simulink model "Bossi_Emanuele_EE460S3D_R99"  (R2025a)
settings: Solver=FixedStepDiscrete  StartTime=0.0  StopTime=120  FixedStep=dt0  RelTol=1e-3  EnableMultiTasking=on
PostLoadFcn:
  | %Set the size for the model
  | set_param(gcs,'Location',[10 10 1270 970])
  | %Set the zoom factor for the model
  | set_param(gcs,'ZoomFactor','100')
InitFcn:
  | tic
  | Bossi_Emanuele_EE460_Final
  | INIT_S3D_01
StartFcn:
  | tend0=toc;
  | tic;
StopFcn:
  | tend=toc;
  | disp(['Simulation time = ' num2str(tout(end)) ' sec'])
  | disp(['Real time = ' num2str(tend) ' sec'])
  | title('DONE')
  | SCORE=round((max(0,120-tout(end)-tend0))*4+10*(40-FuelBurned)+sum(100*double(PDONE)-100*double(PDONE<.5)));
  | PlotS3D(PlotInput);
  | text(15,22,['S: ' num2str(SCORE)]);
  | % Reset color scheme back to normal defaults
  | figure()
  | blkwhitebg('w');
  | close
values from neighbouring files (symbols this model uses):
  A_obs = [ 0  1  0  0  0  0 ... (first row only)    [Bossi_Emanuele_EE460_Final.m]
  B_obs = [ 0     0     0 ... (first row only)    [Bossi_Emanuele_EE460_Final.m]
  C_obs = [ 1 0 0 0 0 0 ... (first row only)    [Bossi_Emanuele_EE460_Final.m]
  d2r = pi/180    (= 0.0174532925199)    [INIT_S3D_01.m]
  D_obs = [ 0     0     0 ... (first row only)    [Bossi_Emanuele_EE460_Final.m]
  dt = 0.01    [INIT_S3D_01.m]
  dt0 = 0.001    [INIT_S3D_01.m]
  fr = 100    [INIT_S3D_01.m]
  G = [1,  1, -1, -1,  0,  0,  0,  0 ... (first row only)    [Bossi_Emanuele_EE460_Final.m]
  G_obs = eye(6)    [Bossi_Emanuele_EE460_Final.m]
  HM_S = 250    [INIT_S3D_01.m]
  HM_U = 500    [INIT_S3D_01.m]
  J = Jbase+JC0+JF+M*(Xcg^2+Ycg^2)    [INIT_S3D_01.m]
  Jbase = JC1+4*Ja+2*Ma*da^2+2*Ma*db^2    [INIT_S3D_01.m]
  JC0 = MC0/2    (= 10.2101761242)    [INIT_S3D_01.m]
  Kdtheta = 2 * zeta_th * wn_th * J_eff    [Bossi_Emanuele_EE460_Final.m]
  Kdtheta_fail = 2 * zeta_th_fail * wn_th_fail * J_eff    [Bossi_Emanuele_EE460_Final.m]
  Kdx = 2 * zeta_xy * wn_xy * M_eff    [Bossi_Emanuele_EE460_Final.m]
  Kdx_fail = 2 * zeta_xy_fail * wn_xy_fail * M_eff    [Bossi_Emanuele_EE460_Final.m]
  Kdy = 2 * zeta_xy * wn_xy * M_eff    [Bossi_Emanuele_EE460_Final.m]
  Kdy_fail = 2 * zeta_xy_fail * wn_xy_fail * M_eff    [Bossi_Emanuele_EE460_Final.m]
  Kptheta = J_eff * wn_th^2    [Bossi_Emanuele_EE460_Final.m]
  Kptheta_fail = J_eff * wn_th_fail^2    [Bossi_Emanuele_EE460_Final.m]
  Kpx = M_eff * wn_xy^2    [Bossi_Emanuele_EE460_Final.m]
  Kpx_fail = M_eff * wn_xy_fail^2    [Bossi_Emanuele_EE460_Final.m]
  Kpy = M_eff * wn_xy^2    [Bossi_Emanuele_EE460_Final.m]
  Kpy_fail = M_eff * wn_xy_fail^2    [Bossi_Emanuele_EE460_Final.m]
  L13 = sqrt(10)    [INIT_S3D_01.m]
  L24 = sqrt(6.25)    [INIT_S3D_01.m]
  LVL = LVL12    [INIT_S3D_01.m]
  M = MC+M1+M2+M3+M4+4*Ma    [INIT_S3D_01.m]
  M1 = LVL.M1    [INIT_S3D_01.m]
  M2 = LVL.M2    [INIT_S3D_01.m]
  M3 = LVL.M3    [INIT_S3D_01.m]
  M4 = LVL.M4    [INIT_S3D_01.m]
  max_qddot = [max_qddot_x; max_qddot_y; max_qddot_theta]    [Bossi_Emanuele_EE460_Final.m]
  mdti = (1/300)    (= 0.00333333333333)    [INIT_S3D_01.m]
  P = [1  1 -1 -1  0  0  0  0 ... (first row only)    [Bossi_Emanuele_EE460_Final.m]
  Pdata = [LVL.P1 LVL.P2 LVL.P3 LVL.P4]    [INIT_S3D_01.m]    (also in PlotS3D.m = R*[xt1;yt1+[0 3*tt*TV(idx-13)*TSIG(idx-13) 0]])
  PTvec = [Pdata(:,1);Pdata(:,2);Pdata(:,3);Pdata(:,4) ... (first row only)    [INIT_S3D_01.m]
  Q_obs = eye(6)    [Bossi_Emanuele_EE460_Final.m]
  r2d = 180/pi    (= 57.2957795131)    [INIT_S3D_01.m]
  r_bang = 0.5    [Bossi_Emanuele_EE460_Final.m]
  Sconfig = 1    [Bossi_Emanuele_EE460_Final.m]
  SLIM = [-100 100 ... (first row only)    [INIT_S3D_01.m]
  SQ = [.005 .01 .004 .005 .01 .004 .02 .01 .4]'    [INIT_S3D_01.m]
  SSF = 1./SQ    [INIT_S3D_01.m]
  tau = 0.5    [Bossi_Emanuele_EE460_Final.m]
  TOLdata = [LVL.P1tol LVL.P2tol LVL.P3tol LVL.P4tol]    [INIT_S3D_01.m]
  ULIM = [[Umin Umax];0 0;0 0]    [INIT_S3D_01.m]
undefined symbols (not defined in the file or in its folder): den_lp, den_lp2, DiscIntNeverNeededParam, dt1_bang_3, dt2_bang_3, dtc_bang_3, num_lp, num_lp2, q0_1
libraries: simulink x87, matrix_library x4, sl3dlib x1, aerolibutil x1, aerolibanimutils x1
(part 1 of 8)
settings Model: Creator=bordignk  LastModifiedBy=emab0
settings SolverCC: AlgebraicLoopSolver=TrustRegion
settings DataIOCC: LimitDataPoints=on  SaveFormat=Array  ReturnWorkspaceOutputs=off
settings OptimizationCC: LifeSpan=inf
settings DebuggingCC: CheckSSInitialOutputMsg=off  UnderspecifiedInitializationDetection=Classic  MergeDetectMultiDrivingBlocksExec=none  InheritedTsInSrcMsg=none  ParameterPrecisionLossMsg=none  AllowSymbolicDim=off  StateNameClashWarn=warning  SFUnexpectedBacktrackingDiag=warning  SFNoUnconditionalDefaultTransitionDiag=warning  SFExecutionAtInitializationDiag=none  ArithmeticOperatorsInVariantConditions=warning
settings HardwareCC: ProdBitPerPointer=32.0  ProdBitPerSizeT=32.0  ProdBitPerPtrDiffT=32.0  ProdLargestAtomicFloat=None  ProdIntDivRoundTo=Undefined  ProdEndianess=Unspecified  ProdWordSize=32.0  ProdHWDeviceType=32-bit Generic
settings ModelReferenceCC: EnableRefExpFcnMdlSchedulingChecks=on  PropagateSignalLabelsOutOfModel=off
settings SFSimCC: SimUseLocalCustomCode=off  CustomCodeUndefinedFunction=UseInterfaceOnly
settings RTWCC: RTWUseLocalCustomCode=off  GPUComputeCapability=3.5  DLArmComputeVersion=19.05
settings CodeAppCC: StateflowObjectComments=on
settings GRTTargetCC: TargetLangStandard=C89/C90 (ANSI)
settings ConfigComp: CovMetricSettings=dw  CovSaveCumulativeToWorkspaceVar=on  CovSaveSingleToWorkspaceVar=on  CovExternalEMLEnable=off

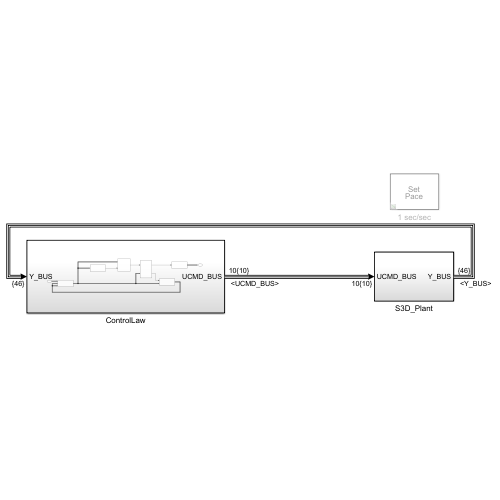
[thumbnail: Simulink's stored preview of the top-level diagram]
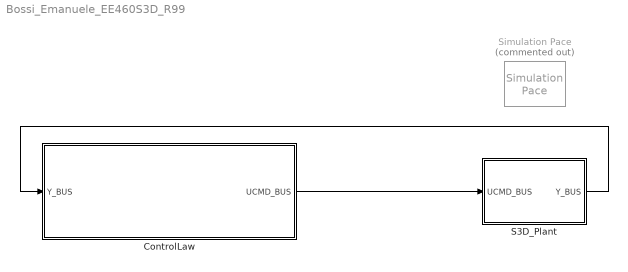
== system Bossi_Emanuele_EE460S3D_R99 ==
  ControlLaw : Subsystem
  S3D_Plant : Subsystem
  Simulation Pace : aerolibanimutils/Simulation Pace  Commented=on  SimulationPace=1  SleepMode=MATLAB Thread  OutputPaceError=off  SampleTime=-1
      settings: AttributesFormatString=%<SimulationPace> sec/sec
  wires:
  S3D_Plant/1(Y_BUS) -> ControlLaw/1(Y_BUS)
  ControlLaw/1(UCMD_BUS) -> S3D_Plant/1(UCMD_BUS)

== system Bossi_Emanuele_EE460S3D_R99/ControlLaw ==
  Y_BUS : Inport
  Command : Subsystem
  ControlAllocation : Subsystem
  InputDataConditioning : Subsystem
  Observer : Subsystem
  OutputDataConditioning : Subsystem
  Regulator : Subsystem
  UCMD_BUS : Outport
  wires:
  OutputDataConditioning/1(UCMD_BUS) -> UCMD_BUS/1
  Y_BUS/1 -> InputDataConditioning/1(Y_BUS)
  ControlAllocation/1(U_lim) -> OutputDataConditioning/1(U_lim)
  Regulator/1(uP_cmd) -> ControlAllocation/1(uP_cmd)
  InputDataConditioning/1(Y_IN) -> Observer/2(Y_IN), ControlAllocation/2(Y_IN), Regulator/1(Y_IN), Command/1(Y_IN)
  ControlAllocation/2(CAout) -> Observer/1(CAout)  "CAout"
  Observer/1(xhat) -> InputDataConditioning/3(xhat_2), InputDataConditioning/2(xhat)  "xhat"
  Command/1(CMD) -> Regulator/2(CMD)  "CMD"

== system Bossi_Emanuele_EE460S3D_R99/S3D_Plant ==
  UCMD_BUS : Inport
  Comm : Subsystem
  GetAccel : Subsystem
  Integrate : Subsystem
  MassProperties : Subsystem
  OutputDataProcessing : Subsystem
  Sensors : Subsystem
  ThrusterValues : Subsystem
  Y_BUS : Outport
  wires:
  Integrate/1(XCentroid) -> OutputDataProcessing/4(x), Comm/1(X), Sensors/1(X), GetAccel/3(X)
  MassProperties/1(MP) -> OutputDataProcessing/1(MP), Integrate/1(MP), GetAccel/1(MP), ThrusterValues/1(MP)
  OutputDataProcessing/1(Y_BUS) -> Y_BUS/1
  Comm/1(COMM) -> OutputDataProcessing/3(COMM)
  Sensors/1(Sensors) -> OutputDataProcessing/2(Sensors)
  ThrusterValues/1(U) -> MassProperties/1(U), OutputDataProcessing/5(U), GetAccel/2(U)
  GetAccel/1(ACCEL) -> Integrate/2(ACCEL)
  UCMD_BUS/1 -> ThrusterValues/2(UCMD_BUS)

== system Bossi_Emanuele_EE460S3D_R99/ControlLaw/Command ==
  Y_IN : Inport
  AutoMode : Subsystem  TreatAsAtomicUnit=on
  Bus Creator : BusCreator  Inputs=6
  Bus Selector : BusSelector  OutputSignals=ManualMode,AutoON,ManualON
  Bus Selector1 : BusSelector  OutputSignals=PointToGo
  Bus Selector2 : BusSelector  OutputSignals=ManualInput
  Bus Selector3 : BusSelector  OutputSignals=Y_IN
  Bus Selector4 : BusSelector  OutputSignals=AutoON,Y_IN
  Bus Selector5 : BusSelector  OutputSignals=ManualMode,Y_IN
  If1 : If  NumInputs=3  IfExpression=u1 == 0 & u2 == 0 & u3 == 0  ElseIfExpressions="(u2  ~= 0 | u3  ~= 0) & u1 == 0"
  InitialPoint : Subsystem  TreatAsAtomicUnit=on
  Joystick : Subsystem
  ManualMode : Subsystem  TreatAsAtomicUnit=on
  Merge : Merge  Inputs=3
  Trigger1 : Subsystem
  Trigger2 : Subsystem
  CMD : Outport
  wires:
  Joystick/1(Out2) -> Bus Creator/1
  Joystick/3(Out4) -> Bus Creator/3  "ManualInput"
  Y_IN/1 -> Bus Creator/6, Joystick/1(Y_IN)
  Joystick/2(Out3) -> Bus Creator/2
  Bus Creator/1 -> Bus Selector2/1, Bus Selector5/1, Bus Selector3/1, Bus Selector1/1, Bus Selector/1, Bus Selector4/1
  Bus Selector1/1 -> AutoMode/1(In2)  "<PointToGo>"
  Merge/1 -> CMD/1  "CMD"
  Bus Selector2/1 -> ManualMode/1(ManualInput)  "<ManualInput>"
  Joystick/4(Out1) -> Bus Creator/4
  ManualMode/1(Out1) -> Merge/3
  AutoMode/1(Out1) -> Merge/2  "CMD"
  InitialPoint/1(Out2) -> Merge/1  "CMD"
  If1/1 -> InitialPoint/Action
  If1/2 -> AutoMode/Action
  If1/3 -> ManualMode/Action
  Bus Selector3/1 -> AutoMode/2(In1)  "<Y_IN>"
  Joystick/5(Out5) -> Bus Creator/5
  Bus Selector/1 -> If1/1  "<ManualMode>"
  Bus Selector/2 -> If1/2  "<AutoON>"
  Bus Selector/3 -> If1/3  "<ManualON>"
  Trigger1/2(Out1) -> InitialPoint/2(In2)
  Bus Selector4/2 -> Trigger1/2(In1)  "<Y_IN>"
  Trigger1/1(Trigger) -> InitialPoint/1(Trigger)
  Bus Selector4/1 -> Trigger1/1(In2)  "<AutoON>"
  Bus Selector5/1 -> Trigger2/1(In2)  "<ManualMode>"
  Bus Selector5/2 -> Trigger2/2(In1)  "<Y_IN>"
  Trigger2/1(Trigger) -> ManualMode/2(Trigger)
  Trigger2/2(TriggeredPosition) -> ManualMode/3(CurrentPosition)
  Trigger2/3(TriggeredVelocity) -> ManualMode/4(CurrentVelocity)

== system Bossi_Emanuele_EE460S3D_R99/ControlLaw/ControlAllocation ==
  uP_cmd : Inport
  Y_IN : Inport  Port=2
  A : Subsystem
  BodyAxisModeling : Subsystem
  Bus Creator : BusCreator  Inputs=2
  Bus Creator1 : BusCreator  Inputs=3
  Bus Selector : BusSelector  OutputSignals=theta_pos_deg
  Bus Selector1 : BusSelector  OutputSignals=R,u_body
  Bus Selector2 : BusSelector  OutputSignals=Failures
  Bus Selector3 : BusSelector  OutputSignals=2A
  Bus Selector4 : BusSelector  OutputSignals=Ufail_mod
  Gain : Gain  Gain=G  Multiplication=Matrix(K*u)
  MatrixMultiply : Product  Multiplication=Matrix(*)
  MatrixMultiply2 : Product  Multiplication=Matrix(*)
  R_theta : Subsystem
  Saturation : Saturate  UpperLimit=100  LowerLimit=0
  Sum : Sum  Inputs=-+|
  Sum1 : Sum  Inputs=++|
  ThrusterFailure : Subsystem
  deg2rad_gain : Gain  Gain=pi/180
  U_lim : Outport  PortDimensions=8
  CAout : Outport  Port=2
  wires:
  MatrixMultiply2/1 -> Sum1/2  "U_mat"
  Saturation/1 -> Gain/1, U_lim/1  "U_lim"
  uP_cmd/1 -> BodyAxisModeling/1(uP_cmd)
  Bus Selector/1 -> deg2rad_gain/1  "<theta_pos_deg>"
  deg2rad_gain/1 -> R_theta/1(In2), BodyAxisModeling/2(theta_rad)  "theta_pos_rad"
  BodyAxisModeling/1(Out1) -> Sum/2  "uP_body"
  MatrixMultiply/1 -> CAout/1  "CAOut"
  R_theta/1(Out1) -> Bus Creator/2  "R"
  Gain/1 -> Bus Creator/1  "u_body"
  Bus Creator/1 -> Bus Selector1/1
  Bus Selector1/1 -> MatrixMultiply/1  "<R>"
  Bus Selector1/2 -> MatrixMultiply/2  "<u_body>"
  Y_IN/1 -> Bus Selector/1, A/1(Y_IN), ThrusterFailure/1(Y_IN)
  A/1(Out1) -> Bus Creator1/1
  Sum/1 -> MatrixMultiply2/2
  ThrusterFailure/1(Out1) -> Bus Creator1/2
  ThrusterFailure/2(Out2) -> Bus Creator1/3
  Bus Creator1/1 -> Bus Selector2/1, Bus Selector3/1, Bus Selector4/1
  Bus Selector2/1 -> Sum/1  "<Failures>"
  Bus Selector3/1 -> MatrixMultiply2/1  "<2A>"
  Sum1/1 -> Saturation/1
  Bus Selector4/1 -> Sum1/1  "<Ufail_mod>"

== system Bossi_Emanuele_EE460S3D_R99/ControlLaw/InputDataConditioning ==
  Y_BUS : Inport
  xhat : Inport  Port=2
  xhat_2 : Inport  Port=3
  Bus Creator : BusCreator  Inputs=55
  Bus Creator1 : BusCreator  Inputs=9
  Bus Selector : BusSelector  OutputSignals=Sensor1,Sensor2,Sensor3,Sensor4,Sensor5,Sensor6,Sensor7,Sensor8,Sensor9
  Bus Selector1 : BusSelector  OutputSignals=P1OK,P1Done,P2OK,P2Done,P3OK,P3Done,P4OK,P4Done
  Bus Selector2 : BusSelector  OutputSignals=Xpos_m,Xvel_mps,Xacc_mps2,Ypos_m,Yvel_mps,Yacc_mps2,theta_pos_deg,theta_vel_degps,theta_acc_degreeps2
  Bus Selector3 : BusSelector  OutputSignals=x_m,xdot_mps,xddot_mps2,y_m,ydot_mps,yddot_mps2,theta_deg,thetadot_degps,thetaddot_degps2
  Bus Selector4 : BusSelector  OutputSignals=S1fail,S2fail,S3fail,S4fail,S5fail,S6fail,S7fail,S8fail,S9fail
  Bus Selector5 : BusSelector  OutputSignals=U1est,U2est,U3est,U4est,U5est,U6est,U7est,U8est,U9est,U10est,U1fail,U2fail,U3fail,U4fail,U5fail,U6fail,U7fail,U8fail,U9fail,U10fail
  Bus Selector6 : BusSelector  OutputSignals=S1fail,S2fail,S3fail,S4fail,S5fail,S6fail,S7fail,S8fail,S9fail
  Mux : Mux  Inputs=9
  Sconfig1 : Subsystem
  Y_IN : Outport
  wires:
  Y_BUS/1 -> Bus Selector6/1, Bus Selector1/1, Bus Selector4/1, Bus Selector5/1, Bus Selector/1
  Bus Selector/1 -> Mux/1  "<Sensor1>"
  Bus Selector/2 -> Mux/2  "<Sensor2>"
  Bus Selector/3 -> Mux/3  "<Sensor3>"
  Bus Selector/4 -> Mux/4  "<Sensor4>"
  Bus Selector/5 -> Mux/5  "<Sensor5>"
  Bus Selector/6 -> Mux/6  "<Sensor6>"
  Bus Selector/7 -> Mux/7  "<Sensor7>"
  Bus Selector/8 -> Mux/8  "<Sensor8>"
  Bus Selector/9 -> Mux/9  "<Sensor9>"
  Mux/1 -> Sconfig1/1(Sensors)  "Sensors"
  Sconfig1/1(Y_IN) -> Bus Selector2/1
  Bus Selector2/1 -> Bus Creator/1  "<Xpos_m>"
  Bus Selector2/2 -> Bus Creator/2  "<Xvel_mps>"
  Bus Selector2/3 -> Bus Creator/3  "<Xacc_mps2>"
  Bus Selector2/4 -> Bus Creator/4  "<Ypos_m>"
  Bus Selector2/5 -> Bus Creator/5  "<Yvel_mps>"
  Bus Selector2/6 -> Bus Creator/6  "<Yacc_mps2>"
  Bus Selector2/7 -> Bus Creator/7  "<theta_pos_deg>"
  Bus Selector2/8 -> Bus Creator/8  "<theta_vel_degps>"
  Bus Selector2/9 -> Bus Creator/9  "<theta_acc_degreeps2>"
  Bus Selector1/1 -> Bus Creator/10  "<P1OK>"
  Bus Selector1/2 -> Bus Creator/11  "<P1Done>"
  Bus Selector1/3 -> Bus Creator/12  "<P2OK>"
  Bus Selector1/4 -> Bus Creator/13  "<P2Done>"
  Bus Selector1/5 -> Bus Creator/14  "<P3OK>"
  Bus Selector1/6 -> Bus Creator/15  "<P3Done>"
  Bus Selector1/7 -> Bus Creator/16  "<P4OK>"
  Bus Selector1/8 -> Bus Creator/17  "<P4Done>"
  Bus Creator/1 -> Y_IN/1  "Y_IN"
  xhat/1 -> Bus Selector3/1
  Bus Selector3/1 -> Bus Creator/18  "<x_m>"
  Bus Selector3/2 -> Bus Creator/19  "<xdot_mps>"
  Bus Selector3/3 -> Bus Creator/20  "<xddot_mps2>"
  Bus Selector3/4 -> Bus Creator/21  "<y_m>"
  Bus Selector3/5 -> Bus Creator/22  "<ydot_mps>"
  Bus Selector3/6 -> Bus Creator/23  "<yddot_mps2>"
  Bus Selector3/7 -> Bus Creator/24  "<theta_deg>"
  Bus Selector3/8 -> Bus Creator/25  "<thetadot_degps>"
  Bus Selector3/9 -> Bus Creator/26  "<thetaddot_degps2>"
  Bus Selector4/1 -> Bus Creator/27  "<S1fail>"
  Bus Selector4/2 -> Bus Creator/28  "<S2fail>"
  Bus Selector4/3 -> Bus Creator/29  "<S3fail>"
  Bus Selector4/4 -> Bus Creator/30  "<S4fail>"
  Bus Selector4/5 -> Bus Creator/31  "<S5fail>"
  Bus Selector4/6 -> Bus Creator/32  "<S6fail>"
  Bus Selector4/7 -> Bus Creator/33  "<S7fail>"
  Bus Selector4/8 -> Bus Creator/34  "<S8fail>"
  Bus Selector4/9 -> Bus Creator/35  "<S9fail>"
  Bus Selector5/1 -> Bus Creator/36  "<U1est>"
  Bus Selector5/2 -> Bus Creator/37  "<U2est>"
  Bus Selector5/3 -> Bus Creator/38  "<U3est>"
  Bus Selector5/4 -> Bus Creator/39  "<U4est>"
  Bus Selector5/5 -> Bus Creator/40  "<U5est>"
  Bus Selector5/6 -> Bus Creator/41  "<U6est>"
  Bus Selector5/7 -> Bus Creator/42  "<U7est>"
  Bus Selector5/8 -> Bus Creator/43  "<U8est>"
  Bus Selector5/9 -> Bus Creator/44  "<U9est>"
  Bus Selector5/10 -> Bus Creator/45  "<U10est>"
  Bus Selector5/11 -> Bus Creator/46  "<U1fail>"
  Bus Selector5/12 -> Bus Creator/47  "<U2fail>"
  Bus Selector5/13 -> Bus Creator/48  "<U3fail>"
  Bus Selector5/14 -> Bus Creator/49  "<U4fail>"
  Bus Selector5/15 -> Bus Creator/50  "<U5fail>"
  Bus Selector5/16 -> Bus Creator/51  "<U6fail>"
  Bus Selector5/17 -> Bus Creator/52  "<U7fail>"
  Bus Selector5/18 -> Bus Creator/53  "<U8fail>"
  Bus Selector5/19 -> Bus Creator/54  "<U9fail>"
  Bus Selector5/20 -> Bus Creator/55  "<U10fail>"
  xhat_2/1 -> Sconfig1/2(xhat_2)
  Bus Selector6/1 -> Bus Creator1/1  "<S1fail>"
  Bus Selector6/2 -> Bus Creator1/2  "<S2fail>"
  Bus Selector6/3 -> Bus Creator1/3  "<S3fail>"
  Bus Selector6/4 -> Bus Creator1/4  "<S4fail>"
  Bus Selector6/5 -> Bus Creator1/5  "<S5fail>"
  Bus Selector6/6 -> Bus Creator1/6  "<S6fail>"
  Bus Selector6/7 -> Bus Creator1/7  "<S7fail>"
  Bus Selector6/8 -> Bus Creator1/8  "<S8fail>"
  Bus Selector6/9 -> Bus Creator1/9  "<S9fail>"
  Bus Creator1/1 -> Sconfig1/3(SensorFailures)

== system Bossi_Emanuele_EE460S3D_R99/ControlLaw/Observer ==
  CAout : Inport
  Y_IN : Inport  Port=2
  Bus Creator : BusCreator  Inputs=6
  Bus Creator1 : BusCreator  Inputs=6
  Bus Creator2 : BusCreator  Inputs=2
  Bus Creator3 : BusCreator  Inputs=9
  Bus Creator4 : BusCreator  Inputs=9
  Bus Selector : BusSelector  OutputSignals=X.x_m,X.xdot_mps,Xdot.xddot_mps2,X.y_m,X.ydot_mps,Xdot.yddot_mps2,X.theta_deg,X.thetadot_degps,Xdot.thetaddot_degps2
  Bus Selector1 : BusSelector  OutputSignals=Xpos_m,Xvel_mps,Xacc_mps2,Ypos_m,Yvel_mps,Yacc_mps2,theta_pos_deg,theta_vel_degps,theta_acc_degreeps2
  Demux : Demux  Outputs=6
  Demux1 : Demux  Outputs=6
  InternalObserver : Subsystem
  Scope : Scope  NumInputPorts=2
      settings: ActiveDisplayYMinimum=-4.6174037693816627  ActiveDisplayYMaximum=4.5675845461186446
  SensorFailureHandling : Subsystem
  xhat : Outport
  wires:
  CAout/1 -> SensorFailureHandling/1(CAout)
  Y_IN/1 -> Bus Selector1/1, SensorFailureHandling/2(Y_IN)
  InternalObserver/1(xdot_hat) -> Demux/1
  InternalObserver/2(x_hat) -> Demux1/1
  Demux/1 -> Bus Creator/1  "xdot_mps"
  Demux/2 -> Bus Creator/2  "xddot_mps2"
  Demux/3 -> Bus Creator/3  "ydot_mps"
  Demux/4 -> Bus Creator/4  "yddot_mps2"
  Demux/5 -> Bus Creator/5  "thetadot_degps"
  Demux/6 -> Bus Creator/6  "thetaddot_degps2"
  Demux1/1 -> Bus Creator1/1  "x_m"
  Demux1/2 -> Bus Creator1/2  "xdot_mps"
  Demux1/3 -> Bus Creator1/3  "y_m"
  Demux1/4 -> Bus Creator1/4  "ydot_mps"
  Demux1/5 -> Bus Creator1/5  "theta_deg"
  Demux1/6 -> Bus Creator1/6  "thetadot_degps"
  Bus Creator/1 -> Bus Creator2/1  "Xdot"
  Bus Creator1/1 -> Bus Creator2/2  "X"
  Bus Creator2/1 -> Bus Selector/1
  Bus Selector/1 -> Bus Creator3/1  "<x_m>"
  Bus Selector/2 -> Bus Creator3/2  "<xdot_mps>"
  Bus Selector/3 -> Bus Creator3/3  "<xddot_mps2>"
  Bus Selector/4 -> Bus Creator3/4  "<y_m>"
  Bus Selector/5 -> Bus Creator3/5  "<ydot_mps>"
  Bus Selector/6 -> Bus Creator3/6  "<yddot_mps2>"
  Bus Selector/7 -> Bus Creator3/7  "<theta_deg>"
  Bus Selector/8 -> Bus Creator3/8  "<thetadot_degps>"
  Bus Selector/9 -> Bus Creator3/9  "<thetaddot_degps2>"
  Bus Creator3/1 -> Scope/1, xhat/1  "xhat"
  SensorFailureHandling/1(Out1) -> InternalObserver/1(CAout)
  SensorFailureHandling/2(Out2) -> InternalObserver/2(Y_IN)
  Bus Selector1/1 -> Bus Creator4/1  "<Xpos_m>"
  Bus Selector1/2 -> Bus Creator4/2  "<Xvel_mps>"
  Bus Selector1/3 -> Bus Creator4/3  "<Xacc_mps2>"
  Bus Selector1/4 -> Bus Creator4/4  "<Ypos_m>"
  Bus Selector1/5 -> Bus Creator4/5  "<Yvel_mps>"
  Bus Selector1/6 -> Bus Creator4/6  "<Yacc_mps2>"
  Bus Selector1/7 -> Bus Creator4/7  "<theta_pos_deg>"
  Bus Selector1/8 -> Bus Creator4/8  "<theta_vel_degps>"
  Bus Selector1/9 -> Bus Creator4/9  "<theta_acc_degreeps2>"
  Bus Creator4/1 -> Scope/2

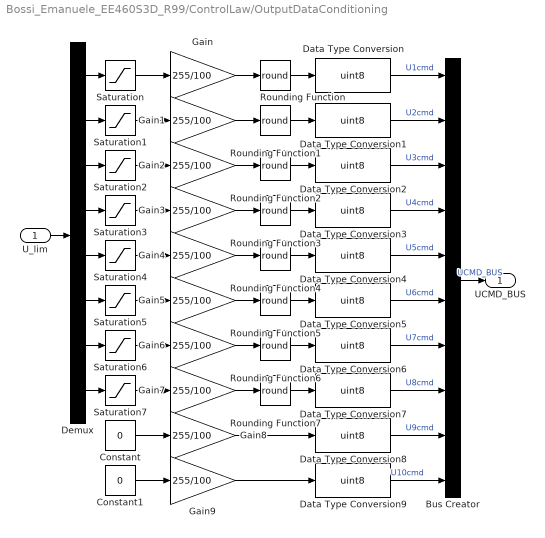
== system Bossi_Emanuele_EE460S3D_R99/ControlLaw/OutputDataConditioning ==
  U_lim : Inport
  Bus Creator : BusCreator  Inputs=10
  Constant : Constant  Value=0
  Constant1 : Constant  Value=0
  Data Type Conversion{,1..9} (10 alike) : DataTypeConversion  OutDataTypeStr=uint8  SaturateOnIntegerOverflow=off  RndMeth=Floor
  Demux : Demux  Outputs=8
  Gain{,1..9} (10 alike) : Gain  Gain=255/100
  Rounding Function{,1..7} (8 alike) : Rounding  Operator=round
  Saturation{,1..7} (8 alike) : Saturate  UpperLimit=100  LowerLimit=0
  UCMD_BUS : Outport
  wires:
  U_lim/1 -> Demux/1
  Demux/1 -> Saturation/1
  Saturation/1 -> Gain/1
  Gain/1 -> Rounding Function/1
  Rounding Function/1 -> Data Type Conversion/1
  Saturation1/1 -> Gain1/1
  Demux/2 -> Saturation1/1
  Gain1/1 -> Rounding Function1/1
  Rounding Function1/1 -> Data Type Conversion1/1
  Saturation2/1 -> Gain2/1
  Demux/3 -> Saturation2/1
  Gain2/1 -> Rounding Function2/1
  Rounding Function2/1 -> Data Type Conversion2/1
  Saturation3/1 -> Gain3/1
  Demux/4 -> Saturation3/1
  Gain3/1 -> Rounding Function3/1
  Rounding Function3/1 -> Data Type Conversion3/1
  Saturation4/1 -> Gain4/1
  Demux/5 -> Saturation4/1
  Gain4/1 -> Rounding Function4/1
  Rounding Function4/1 -> Data Type Conversion4/1
  Gain5/1 -> Rounding Function5/1
  Saturation5/1 -> Gain5/1
  Rounding Function5/1 -> Data Type Conversion5/1
  Demux/6 -> Saturation5/1
  Gain6/1 -> Rounding Function6/1
  Saturation6/1 -> Gain6/1
  Rounding Function6/1 -> Data Type Conversion6/1
  Demux/7 -> Saturation6/1
  Gain7/1 -> Rounding Function7/1
  Saturation7/1 -> Gain7/1
  Rounding Function7/1 -> Data Type Conversion7/1
  Demux/8 -> Saturation7/1
  Data Type Conversion/1 -> Bus Creator/1  "U1cmd"
  Data Type Conversion1/1 -> Bus Creator/2  "U2cmd"
  Data Type Conversion2/1 -> Bus Creator/3  "U3cmd"
  Data Type Conversion3/1 -> Bus Creator/4  "U4cmd"
  Data Type Conversion4/1 -> Bus Creator/5  "U5cmd"
  Data Type Conversion5/1 -> Bus Creator/6  "U6cmd"
  Data Type Conversion6/1 -> Bus Creator/7  "U7cmd"
  Data Type Conversion7/1 -> Bus Creator/8  "U8cmd"
  Data Type Conversion8/1 -> Bus Creator/9  "U9cmd"
  Data Type Conversion9/1 -> Bus Creator/10  "U10cmd"
  Bus Creator/1 -> UCMD_BUS/1  "UCMD_BUS"
  Constant/1 -> Gain8/1
  Gain8/1 -> Data Type Conversion8/1
  Constant1/1 -> Gain9/1
  Gain9/1 -> Data Type Conversion9/1

== system Bossi_Emanuele_EE460S3D_R99/ControlLaw/Regulator ==
  Y_IN : Inport
  CMD : Inport  Port=2
  Bus Creator : BusCreator  Inputs=17
  Bus Creator1 : BusCreator  Inputs=9
  Bus Selector : BusSelector  OutputSignals=x_m,xdot_mps,y_m,ydot_mps,theta_deg,thetadot_degps,U1fail,U2fail,U3fail,U4fail,U5fail,U6fail,U7fail,U8fail
  Bus Selector1 : BusSelector  OutputSignals=U1fail,U2fail,U3fail,U4fail,U5fail,U6fail,U7fail,U8fail
  Bus Selector2 : BusSelector  OutputSignals=x_cmd,y_cmd,theta_cmd
  Demux : Demux  Outputs=9
  If : If  IfExpression=u1 == 0
  Merge : Merge
  NoFailures : Subsystem  TreatAsAtomicUnit=on
  Sum : Sum  Inputs=++++++++
  ThrusterFailures : Subsystem  TreatAsAtomicUnit=on
  uP_cmd : Outport
  wires:
  CMD/1 -> Demux/1
  Y_IN/1 -> Bus Selector/1
  Bus Selector/1 -> Bus Creator/1  "<x_m>"
  Bus Creator/1 -> ThrusterFailures/1(In1), NoFailures/1(In1), Bus Selector1/1  "vars"
  NoFailures/1(uP_cmd) -> Merge/1  "uP"
  Demux/1 -> Bus Creator1/1  "x_cmd"
  Demux/2 -> Bus Creator1/2  "y_cmd"
  Demux/3 -> Bus Creator1/3  "theta_cmd"
  Demux/4 -> Bus Creator1/4  "xdot_cmd"
  Demux/5 -> Bus Creator1/5  "ydot_cmd"
  Demux/6 -> Bus Creator1/6  "thetadot_cmd"
  Demux/7 -> Bus Creator1/7  "xddot_cmd"
  Demux/8 -> Bus Creator1/8  "yddot_cmd"
  Demux/9 -> Bus Creator1/9  "thetaddot_cmd"
  Bus Creator1/1 -> Bus Selector2/1
  Bus Selector2/1 -> Bus Creator/15  "<x_cmd>"
  Bus Selector2/2 -> Bus Creator/16  "<y_cmd>"
  Bus Selector2/3 -> Bus Creator/17  "<theta_cmd>"
  Bus Selector/2 -> Bus Creator/2  "<xdot_mps>"
  Bus Selector/3 -> Bus Creator/3  "<y_m>"
  Bus Selector/4 -> Bus Creator/4  "<ydot_mps>"
  Bus Selector/5 -> Bus Creator/5  "<theta_deg>"
  Bus Selector/6 -> Bus Creator/6  "<thetadot_degps>"
  Bus Selector/7 -> Bus Creator/7  "<U1fail>"
  Bus Selector/8 -> Bus Creator/8  "<U2fail>"
  Bus Selector/9 -> Bus Creator/9  "<U3fail>"
  Bus Selector/10 -> Bus Creator/10  "<U4fail>"
  Bus Selector/11 -> Bus Creator/11  "<U5fail>"
  Bus Selector/12 -> Bus Creator/12  "<U6fail>"
  Bus Selector/13 -> Bus Creator/13  "<U7fail>"
  Bus Selector/14 -> Bus Creator/14  "<U8fail>"
  Bus Selector1/1 -> Sum/1  "<U1fail>"
  Bus Selector1/8 -> Sum/8  "<U8fail>"
  Bus Selector1/7 -> Sum/7  "<U7fail>"
  Bus Selector1/6 -> Sum/6  "<U6fail>"
  Bus Selector1/2 -> Sum/2  "<U2fail>"
  Bus Selector1/3 -> Sum/3  "<U3fail>"
  Bus Selector1/4 -> Sum/4  "<U4fail>"
  Bus Selector1/5 -> Sum/5  "<U5fail>"
  Sum/1 -> If/1
  If/1 -> NoFailures/Action
  If/2 -> ThrusterFailures/Action
  Merge/1 -> uP_cmd/1  "uP"
  ThrusterFailures/1(uP_cmd) -> Merge/2  "uP"

== system Bossi_Emanuele_EE460S3D_R99/S3D_Plant/Comm ==
  X : Inport
  Bus Creator : BusCreator  Inputs=8
  Bus Selector : BusSelector  OutputSignals=P1Done,P2Done,P3Done,P4Done  OutputAsBus=on
  Bus Selector1 : BusSelector  OutputSignals=P1Done,P2Done,P3Done,P4Done  OutputAsBus=on
  Compare To Constant : simulink/Logic and Bit Operations/Compare To Constant  relop=>=  const=4  OutDataTypeStr=boolean
  Data Type Conversion : DataTypeConversion  OutDataTypeStr=uint8  SaturateOnIntegerOverflow=off  RndMeth=Floor
  P1 : Subsystem  mask{Pdx=1}
      mask prompts: Pdx "Data Point (1-4)"
  P2 : Subsystem  mask{Pdx=2}
      mask prompts: Pdx "Data Point (1-4)"
  P3 : Subsystem  mask{Pdx=3}
      mask prompts: Pdx "Data Point (1-4)"
  P4 : Subsystem  mask{Pdx=4}
      mask prompts: Pdx "Data Point (1-4)"
  Stop Simulation : Stop
  Sum of Elements : Sum  Inputs=+
  To Workspace : ToWorkspace  VariableName=PDONE  SampleTime=dt0
      settings: MaxDataPoints=1
  COMM : Outport
  wires:
  Compare To Constant/1 -> Stop Simulation/1
  Sum of Elements/1 -> Compare To Constant/1
  Data Type Conversion/1 -> Sum of Elements/1
  Bus Selector1/1 -> Data Type Conversion/1
  Bus Selector/1 -> To Workspace/1  "PDONE"
  Bus Creator/1 -> COMM/1, Bus Selector/1, Bus Selector1/1  "COMM"
  P4/1(COMM_OK) -> Bus Creator/7  "P4OK"
  P4/2(COMM_DONE) -> Bus Creator/8  "P4Done"
  P3/1(COMM_OK) -> Bus Creator/5  "P3OK"
  P3/2(COMM_DONE) -> Bus Creator/6  "P3Done"
  P2/1(COMM_OK) -> Bus Creator/3  "P2OK"
  P2/2(COMM_DONE) -> Bus Creator/4  "P2Done"
  P1/2(COMM_DONE) -> Bus Creator/2  "P1Done"
  P1/1(COMM_OK) -> Bus Creator/1  "P1OK"
  X/1 -> P3/1(X), P4/1(X), P2/1(X), P1/1(X)

== system Bossi_Emanuele_EE460S3D_R99/S3D_Plant/GetAccel ==
  MP : Inport
  U : Inport  Port=2
  X : Inport  Port=3
  Bus Creator : BusCreator  Inputs=3
  GetFxb : Subsystem
  GetFyb : Subsystem
  GetMz : Subsystem
  InertialAccel : Subsystem
  ACCEL : Outport
  wires:
  InertialAccel/1(ACCEL) -> ACCEL/1
  Bus Creator/1 -> InertialAccel/1(FM)  "FM"
  MP/1 -> GetMz/2(MP), InertialAccel/2(MP)
  X/1 -> InertialAccel/3(X)
  U/1 -> GetFxb/1(U), GetFyb/1(U), GetMz/1(U)
  GetFxb/1(Fxb) -> Bus Creator/1
  GetFyb/1(Fyb) -> Bus Creator/2
  GetMz/1(Mzb) -> Bus Creator/3

== system Bossi_Emanuele_EE460S3D_R99/S3D_Plant/Integrate ==
  MP : Inport
  ACCEL : Inport  Port=2
  ABM_INT1 : Subsystem
  Bus Creator : BusCreator  Inputs=9
  Bus Selector2 : BusSelector  OutputSignals=xddt_mps2,yddt_mps2,thtddt_rps2
  Bus to Vector1 : BusToVector
  CentroidData : Subsystem
  Demux : Demux  Outputs=6
  Mux : Mux  Inputs=2
  Selector : Selector  InputPortWidth=6  IndexOptions=Index vector (dialog)  Indices=[4 5 6]  OutputSizes=1
  XCentroid : Outport
  wires:
  CentroidData/1(XCentroid) -> XCentroid/1
  MP/1 -> CentroidData/1(MP)
  Bus Selector2/3 -> Bus Creator/9  "<thtddt_rps2>"
  Bus Selector2/1 -> Bus Creator/7  "<xddt_mps2>"
  Bus Selector2/2 -> Bus Creator/8  "<yddt_mps2>"
  Bus to Vector1/1 -> Mux/2
  Bus Creator/1 -> CentroidData/2(XCG)  "XCG"
  Selector/1 -> Mux/1
  ACCEL/1 -> Bus to Vector1/1, Bus Selector2/1
  Demux/4 -> Bus Creator/4  "xdt_mps"
  Demux/6 -> Bus Creator/6  "thtdt_rps"
  Demux/5 -> Bus Creator/5  "ydt_mps"
  Demux/2 -> Bus Creator/2  "y_m"
  Demux/1 -> Bus Creator/1  "x_m"
  Demux/3 -> Bus Creator/3  "tht_rad"
  Mux/1 -> ABM_INT1/1(DX)  "DX"
  ABM_INT1/1(X) -> Selector/1, Demux/1

== system Bossi_Emanuele_EE460S3D_R99/S3D_Plant/MassProperties ==
  U : Inport
  Bus Creator : BusCreator  Inputs=6
  Bus Selector : BusSelector  OutputSignals=U1,U2,U3,U4,U5,U6,U7,U8  OutputAsBus=on
  Bus to Vector : BusToVector
  Constant : Constant  Value=[M1 M2 M3 M4]  SampleTime=dt0
  Constant1 : Constant  Value=60  SampleTime=dt0
  Discrete-Time Integrator : DiscreteIntegrator  SampleTime=dt0  UpperSaturationLimit=10  LowerSaturationLimit=0  ICPrevOutput=DiscIntNeverNeededParam  ICPrevScaledInput=DiscIntNeverNeededParam
  Gain1 : Gain  Gain=LVL.FB
  Gain4 : Gain  Gain=mdti
  GetCGnJ : Subsystem
  Mux1 : Mux
  Saturation : Saturate  UpperLimit=10  LowerLimit=0
  Selector : Selector  InputPortWidth=8  IndexOptions=Index vector (dialog)  Indices=[1 5]  OutputSizes=1
  Selector2 : Selector  InputPortWidth=8  IndexOptions=Index vector (dialog)  Indices=[2 6]  OutputSizes=1
  Selector3 : Selector  InputPortWidth=8  IndexOptions=Index vector (dialog)  Indices=[3 7]  OutputSizes=1
  Selector4 : Selector  InputPortWidth=8  IndexOptions=Index vector (dialog)  Indices=[4 8]  OutputSizes=1
  Sum : Sum  Inputs=|+-
  Sum of Elements{,1..5} (6 alike) : Sum  Inputs=+
  Sum1 : Sum  Inputs=|++
  To Workspace : ToWorkspace  VariableName=FuelBurned  SampleTime=dt0
      settings: MaxDataPoints=1
  MP : Outport
  wires:
  Gain1/1 -> Selector/1, Selector2/1, Selector3/1, Selector4/1
  Bus Creator/1 -> MP/1  "MP"
  GetCGnJ/3(J) -> Bus Creator/3
  GetCGnJ/2(Ycg) -> Bus Creator/2
  GetCGnJ/1(Xcg) -> Bus Creator/1
  Sum1/1 -> GetCGnJ/2(M_kg), Bus Creator/4  "M_kg"
  Sum of Elements3/1 -> Bus Creator/5, Sum1/2  "Mfuel_kg"
  Constant1/1 -> Sum1/1
  Saturation/1 -> Sum of Elements3/1, GetCGnJ/1(MfuelVector), Bus Creator/6  "MfuelVector"
  Sum/1 -> Saturation/1
  Constant/1 -> Sum/1
  Bus Selector/1 -> Bus to Vector/1
  U/1 -> Bus Selector/1
  Sum of Elements/1 -> Mux1/1
  Selector4/1 -> Sum of Elements4/1
  Selector3/1 -> Sum of Elements2/1
  Sum of Elements1/1 -> Mux1/2
  Sum of Elements2/1 -> Mux1/3
  Sum of Elements4/1 -> Mux1/4
  Mux1/1 -> Sum/2
  Gain4/1 -> Discrete-Time Integrator/1
  Selector/1 -> Sum of Elements/1
  Selector2/1 -> Sum of Elements1/1
  Bus to Vector/1 -> Gain4/1
  Discrete-Time Integrator/1 -> Sum of Elements5/1, Gain1/1
  Sum of Elements5/1 -> To Workspace/1

== system Bossi_Emanuele_EE460S3D_R99/S3D_Plant/OutputDataProcessing ==
  MP : Inport
  Sensors : Inport  Port=2
  COMM : Inport  Port=3
  x : Inport  Port=4
  U : Inport  Port=5
  Bus Creator1 : BusCreator  Inputs=46
  Bus Selector : BusSelector  OutputSignals=U1,U2,U3,U4,U5,U6,U7,U8,U9,U10,U1fail,U2fail,U3fail,U4fail,U5fail,U6fail,U7fail,U8fail,U9fail,U10fail
  Bus Selector1 : BusSelector  OutputSignals=Sensor1,Sensor2,Sensor3,Sensor4,Sensor5,Sensor6,Sensor7,Sensor8,Sensor9,S1fail,S2fail,S3fail,S4fail,S5fail,S6fail,S7fail,S8fail,S9fail
  Bus Selector2 : BusSelector  OutputSignals=P1OK,P1Done,P2OK,P2Done,P3OK,P3Done,P4OK,P4Done
  Data Type Conversion{,1..9} (10 alike) : DataTypeConversion  OutDataTypeStr=uint8  SaturateOnIntegerOverflow=off  RndMeth=Floor
  MakePlot : Subsystem
  Rate Transition : RateTransition  OutPortSampleTime=dt
  Unit Delay : UnitDelay  SampleTime=dt0  HasFrameUpgradeWarning=on
  Y_BUS : Outport
  wires:
  x/1 -> MakePlot/4(x)
  MP/1 -> MakePlot/3(MP)
  Data Type Conversion9/1 -> Bus Creator1/28  "U10est"
  Data Type Conversion8/1 -> Bus Creator1/27  "U9est"
  Data Type Conversion7/1 -> Bus Creator1/26  "U8est"
  Data Type Conversion6/1 -> Bus Creator1/25  "U7est"
  Data Type Conversion5/1 -> Bus Creator1/24  "U6est"
  Data Type Conversion4/1 -> Bus Creator1/23  "U5est"
  Data Type Conversion3/1 -> Bus Creator1/22  "U4est"
  Data Type Conversion2/1 -> Bus Creator1/21  "U3est"
  Data Type Conversion1/1 -> Bus Creator1/20  "U2est"
  Data Type Conversion/1 -> Bus Creator1/19  "U1est"
  Bus Selector1/16 -> Bus Creator1/16  "<S7fail>"
  Bus Selector1/18 -> Bus Creator1/18  "<S9fail>"
  Bus Selector1/15 -> Bus Creator1/15  "<S6fail>"
  Bus Selector1/14 -> Bus Creator1/14  "<S5fail>"
  Bus Selector1/13 -> Bus Creator1/13  "<S4fail>"
  Bus Selector1/12 -> Bus Creator1/12  "<S3fail>"
  Bus Selector1/11 -> Bus Creator1/11  "<S2fail>"
  Bus Selector1/10 -> Bus Creator1/10  "<S1fail>"
  Bus Selector1/9 -> Bus Creator1/9  "<Sensor9>"
  Bus Selector1/8 -> Bus Creator1/8  "<Sensor8>"
  Bus Selector1/6 -> Bus Creator1/6  "<Sensor6>"
  Bus Selector1/1 -> Bus Creator1/1  "<Sensor1>"
  Bus Selector1/2 -> Bus Creator1/2  "<Sensor2>"
  Bus Selector1/17 -> Bus Creator1/17  "<S8fail>"
  Bus Selector1/3 -> Bus Creator1/3  "<Sensor3>"
  Bus Selector1/4 -> Bus Creator1/4  "<Sensor4>"
  Bus Selector1/5 -> Bus Creator1/5  "<Sensor5>"
  Bus Selector1/7 -> Bus Creator1/7  "<Sensor7>"
  Bus Selector/11 -> Bus Creator1/29  "<U1fail>"
  Bus Selector/16 -> Bus Creator1/34  "<U6fail>"
  Bus Selector/13 -> Bus Creator1/31  "<U3fail>"
  Bus Selector/15 -> Bus Creator1/33  "<U5fail>"
  Bus Selector/20 -> Bus Creator1/38  "<U10fail>"
  Bus Selector/1 -> Data Type Conversion/1  "<U1>"
  Bus Selector/18 -> Bus Creator1/36  "<U8fail>"
  Bus Selector/2 -> Data Type Conversion1/1  "<U2>"
  Bus Selector/19 -> Bus Creator1/37  "<U9fail>"
  Bus Selector/12 -> Bus Creator1/30  "<U2fail>"
  Bus Selector/4 -> Data Type Conversion3/1  "<U4>"
  Bus Selector/17 -> Bus Creator1/35  "<U7fail>"
  Bus Selector/14 -> Bus Creator1/32  "<U4fail>"
  Bus Selector/10 -> Data Type Conversion9/1  "<U10>"
  Bus Selector/8 -> Data Type Conversion7/1  "<U8>"
  Bus Selector/9 -> Data Type Conversion8/1  "<U9>"
  Bus Selector/7 -> Data Type Conversion6/1  "<U7>"
  Bus Selector/6 -> Data Type Conversion5/1  "<U6>"
  Bus Selector/5 -> Data Type Conversion4/1  "<U5>"
  Bus Selector/3 -> Data Type Conversion2/1  "<U3>"
  Rate Transition/1 -> Y_BUS/1  "Y_BUS"
  Unit Delay/1 -> Rate Transition/1
  Bus Selector2/7 -> Bus Creator1/45  "<P4OK>"
  Bus Selector2/4 -> Bus Creator1/42  "<P2Done>"
  Bus Selector2/6 -> Bus Creator1/44  "<P3Done>"
  Bus Selector2/1 -> Bus Creator1/39  "<P1OK>"
  Bus Selector2/2 -> Bus Creator1/40  "<P1Done>"
  Bus Selector2/5 -> Bus Creator1/43  "<P3OK>"
  Bus Selector2/3 -> Bus Creator1/41  "<P2OK>"
  Bus Selector2/8 -> Bus Creator1/46  "<P4Done>"
  COMM/1 -> Bus Selector2/1, MakePlot/5(COMM)
  Sensors/1 -> MakePlot/2(Sensors), Bus Selector1/1
  U/1 -> Bus Selector/1, MakePlot/1(U)
  Bus Creator1/1 -> Unit Delay/1

== system Bossi_Emanuele_EE460S3D_R99/S3D_Plant/Sensors ==
  X : Inport
  CASE1 : Subsystem  TreatAsAtomicUnit=on
  CASE2 : Subsystem  TreatAsAtomicUnit=on
  CASE3 : Subsystem  TreatAsAtomicUnit=on
  Constant : Constant  Value=Sconfig  SampleTime=dt0
  ConvertINT16 : Subsystem
  HealthMonitoring : Subsystem
  Merge : Merge  Inputs=3
  Switch Case : SwitchCase  CaseConditions={1,2}  SampleTime=dt0
  Sensors : Outport
  wires:
  HealthMonitoring/1(Sensors) -> Sensors/1
  ConvertINT16/1(INT16) -> HealthMonitoring/1(SensorValues)
  Merge/1 -> ConvertINT16/1(SDouble)  "SDouble"
  X/1 -> CASE1/1(X), CASE2/1(X), CASE3/1(X)
  CASE3/1(Out1) -> Merge/3
  CASE2/1(Out1) -> Merge/2
  CASE1/1(Out1) -> Merge/1
  Switch Case/3 -> CASE3/Action
  Switch Case/2 -> CASE2/Action
  Switch Case/1 -> CASE1/Action
  Constant/1 -> Switch Case/1

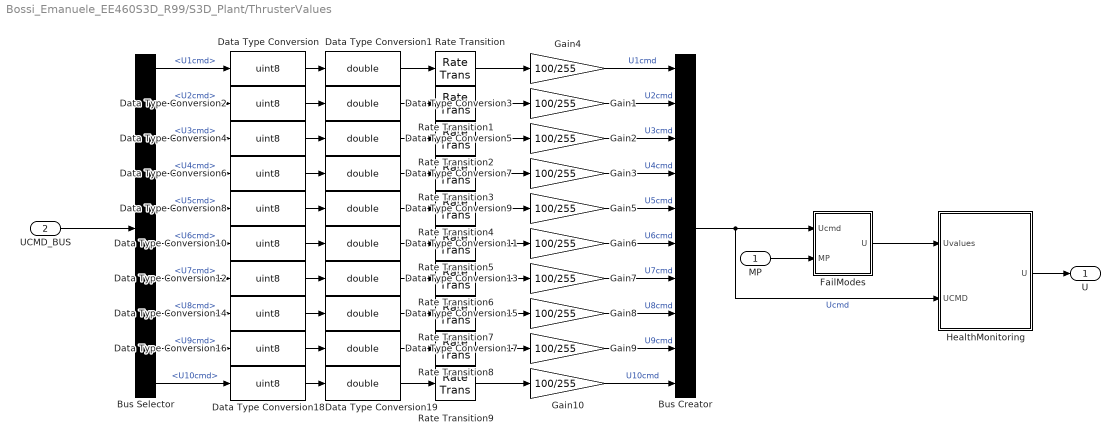
== system Bossi_Emanuele_EE460S3D_R99/S3D_Plant/ThrusterValues ==
  MP : Inport
  UCMD_BUS : Inport  Port=2
  Bus Creator : BusCreator  Inputs=10
  Bus Selector : BusSelector  OutputSignals=U1cmd,U2cmd,U3cmd,U4cmd,U5cmd,U6cmd,U7cmd,U8cmd,U9cmd,U10cmd
  Data Type Conversion{,2,4,6,8,10,12,14,16,18} (10 alike) : DataTypeConversion  OutDataTypeStr=uint8  SaturateOnIntegerOverflow=off  RndMeth=Floor
  Data Type Conversion{1,3,5,7,9,11,13,15,17,19} (10 alike) : DataTypeConversion  OutDataTypeStr=double  SaturateOnIntegerOverflow=off  RndMeth=Floor
  FailModes : Subsystem
  Gain{1..10} (10 alike) : Gain  Gain=100/255
  HealthMonitoring : Subsystem
  Rate Transition{,1..9} (10 alike) : RateTransition  OutPortSampleTime=dt0
  U : Outport
  wires:
  Rate Transition9/1 -> Gain10/1
  Rate Transition8/1 -> Gain9/1
  Rate Transition7/1 -> Gain8/1
  Rate Transition6/1 -> Gain7/1
  Rate Transition5/1 -> Gain6/1
  Rate Transition4/1 -> Gain5/1
  Rate Transition3/1 -> Gain3/1
  Rate Transition2/1 -> Gain2/1
  Rate Transition1/1 -> Gain1/1
  Rate Transition/1 -> Gain4/1
  HealthMonitoring/1(U) -> U/1
  FailModes/1(U) -> HealthMonitoring/1(Uvalues)
  MP/1 -> FailModes/2(MP)
  Gain10/1 -> Bus Creator/10  "U10cmd"
  Gain9/1 -> Bus Creator/9  "U9cmd"
  Bus Selector/10 -> Data Type Conversion18/1  "<U10cmd>"
  Bus Selector/9 -> Data Type Conversion16/1  "<U9cmd>"
  Data Type Conversion19/1 -> Rate Transition9/1
  Data Type Conversion18/1 -> Data Type Conversion19/1
  Data Type Conversion17/1 -> Rate Transition8/1
  Data Type Conversion16/1 -> Data Type Conversion17/1
  Bus Creator/1 -> FailModes/1(Ucmd), HealthMonitoring/2(UCMD)  "Ucmd"
  Gain8/1 -> Bus Creator/8  "U8cmd"
  Gain7/1 -> Bus Creator/7  "U7cmd"
  Gain6/1 -> Bus Creator/6  "U6cmd"
  Gain5/1 -> Bus Creator/5  "U5cmd"
  Gain3/1 -> Bus Creator/4  "U4cmd"
  Gain2/1 -> Bus Creator/3  "U3cmd"
  Gain1/1 -> Bus Creator/2  "U2cmd"
  Gain4/1 -> Bus Creator/1  "U1cmd"
  Bus Selector/8 -> Data Type Conversion14/1  "<U8cmd>"
  Bus Selector/7 -> Data Type Conversion12/1  "<U7cmd>"
  Bus Selector/6 -> Data Type Conversion10/1  "<U6cmd>"
  Bus Selector/5 -> Data Type Conversion8/1  "<U5cmd>"
  Bus Selector/4 -> Data Type Conversion6/1  "<U4cmd>"
  Bus Selector/3 -> Data Type Conversion4/1  "<U3cmd>"
  Data Type Conversion15/1 -> Rate Transition7/1
  Data Type Conversion14/1 -> Data Type Conversion15/1
  Data Type Conversion13/1 -> Rate Transition6/1
  Data Type Conversion12/1 -> Data Type Conversion13/1
  Data Type Conversion11/1 -> Rate Transition5/1
  Data Type Conversion10/1 -> Data Type Conversion11/1
  Data Type Conversion9/1 -> Rate Transition4/1
  Data Type Conversion8/1 -> Data Type Conversion9/1
  Data Type Conversion7/1 -> Rate Transition3/1
  Data Type Conversion6/1 -> Data Type Conversion7/1
  Data Type Conversion5/1 -> Rate Transition2/1
  Data Type Conversion4/1 -> Data Type Conversion5/1
  Bus Selector/2 -> Data Type Conversion2/1  "<U2cmd>"
  Data Type Conversion3/1 -> Rate Transition1/1
  Data Type Conversion2/1 -> Data Type Conversion3/1
  Data Type Conversion1/1 -> Rate Transition/1
  Data Type Conversion/1 -> Data Type Conversion1/1
  Bus Selector/1 -> Data Type Conversion/1  "<U1cmd>"
  UCMD_BUS/1 -> Bus Selector/1

== system Bossi_Emanuele_EE460S3D_R99/ControlLaw/Command/AutoMode ==
  In2 : Inport
  In1 : Inport  Port=2
  Action Port : ActionPort  ActionPortLabel="elseif((u2  ~= 0 | u3  ~= 0) & u1 == 0)"
  BangBang_cmd : Subsystem
  Bus Creator : BusCreator  Inputs=4
  Bus Creator1 : BusCreator  Inputs=3
  Bus Creator2 : BusCreator  Inputs=3
  Bus Creator3 : BusCreator  Inputs=2
  Bus Selector : BusSelector  OutputSignals=Xpos_m,Ypos_m,theta_pos_deg
  Bus Selector1 : BusSelector  OutputSignals=velocities,PointToGo,positions
  Bus Selector2 : BusSelector  OutputSignals=PointToGo
  Bus Selector3 : BusSelector  OutputSignals=Xvel_mps,Yvel_mps,theta_vel_degps
  Bus Selector4 : BusSelector  OutputSignals=Trigger,velocities
  Constant : Constant  Value=Pdata  SampleTime=dt
  FinalPositionSelector : Subsystem
  PositionTrigger : Subsystem  TreatAsAtomicUnit=on
  TriggerCondition : Subsystem
  VelocityTrigger : Subsystem  TreatAsAtomicUnit=on
  Out1 : Outport
  wires:
  BangBang_cmd/1(Out1) -> Out1/1  "CMD"
  In1/1 -> Bus Selector3/1, Bus Selector/1
  Bus Selector/1 -> Bus Creator1/1  "<Xpos_m>"
  Bus Selector/2 -> Bus Creator1/2  "<Ypos_m>"
  Bus Selector/3 -> Bus Creator1/3  "<theta_pos_deg>"
  Bus Creator/1 -> Bus Selector2/1, Bus Selector1/1
  Bus Creator1/1 -> Bus Creator/3  "positions"
  Constant/1 -> Bus Creator/2  "Pdata"
  In2/1 -> Bus Creator/1
  TriggerCondition/1(Trigger) -> PositionTrigger/Trigger, BangBang_cmd/3(Trigger), Bus Creator3/2
  Bus Selector1/2 -> TriggerCondition/1(In2)  "<PointToGo>"
  Bus Selector1/3 -> PositionTrigger/1(In1)  "<positions>"
  Bus Selector2/1 -> FinalPositionSelector/1(In2)  "<PointToGo>"
  PositionTrigger/1(CurrentPosition1) -> BangBang_cmd/4(CurrentPosition1), BangBang_cmd/6(CurrentPosition4), BangBang_cmd/5(CurrentPosition3)
  FinalPositionSelector/1(FinalPosition) -> BangBang_cmd/8(FinalPosition1), BangBang_cmd/7(FinalPosition)
  Bus Selector3/1 -> Bus Creator2/1  "<Xvel_mps>"
  Bus Selector3/2 -> Bus Creator2/2  "<Yvel_mps>"
  Bus Selector3/3 -> Bus Creator2/3  "<theta_vel_degps>"
  Bus Creator2/1 -> Bus Creator/4  "velocities"
  Bus Selector1/1 -> Bus Creator3/1  "<velocities>"
  Bus Creator3/1 -> Bus Selector4/1
  VelocityTrigger/1(CurrentVelocity) -> BangBang_cmd/2(CurrentVelocity), BangBang_cmd/1(In1)
  Bus Selector4/1 -> VelocityTrigger/Trigger  "<Trigger>"
  Bus Selector4/2 -> VelocityTrigger/1(In1)  "<velocities>"

== system Bossi_Emanuele_EE460S3D_R99/ControlLaw/Command/InitialPoint ==
  Trigger : Inport
  In2 : Inport  Port=2
  Action Port : ActionPort  ActionPortLabel=if(u1 == 0 & u2 == 0 & u3 == 0)
  BangBang_cmd : Subsystem
  Out2 : Outport
  wires:
  In2/1 -> BangBang_cmd/3(CurrentPosition3), BangBang_cmd/4(CurrentPosition4), BangBang_cmd/2(CurrentPosition1)
  BangBang_cmd/1(Out1) -> Out2/1  "CMD"
  Trigger/1 -> BangBang_cmd/1(Trigger)

== system Bossi_Emanuele_EE460S3D_R99/ControlLaw/Command/Joystick ==
  Y_IN : Inport
  Bus Creator : BusCreator  Inputs=3
  Constant : Constant  Value=0
  Demux : Demux  Outputs=5
  Demux1 : Demux  Outputs=3
  Display2 : Display
  Hold : Subsystem
  Hold1 : Subsystem
  MissionNum : Subsystem
  PointToGo : Subsystem
  Rate Transition : RateTransition  OutPortSampleTime=dt
  Rate Transition1 : RateTransition  OutPortSampleTime=dt
  Rate Transition2 : RateTransition  OutPortSampleTime=dt
  Saturation : Saturate  UpperLimit=4  LowerLimit=0
  Selector : Selector  IndexOptions=Index vector (dialog)  Indices=[5 6 7 8 9]  OutputSizes=1
  Selector1 : Selector  IndexOptions=Index vector (dialog)  Indices=[1 2 3]  OutputSizes=1
  Selector2 : Selector  IndexOptions=Index vector (dialog)  Indices=[3]  OutputSizes=1
  Simulation 3D Joystick : sl3dlib/Simulation 3D/Hardware Interface/Simulation 3D Joystick  joyid=1  adjustports=on  forcefeed=off
  Switch : Switch  Criteria=u2 > Threshold  SaturateOnIntegerOverflow=off  InputSameDT=off
  Out2 : Outport
  Out3 : Outport  Port=2
  Out4 : Outport  Port=3
  Out1 : Outport  Port=4
  Out5 : Outport  Port=5
  wires:
  Bus Creator/1 -> Out4/1  "ManualInput"
  Hold/1(Out1) -> Out3/1
  Demux1/2 -> Bus Creator/2  "u_y_raw"
  MissionNum/1(Out1) -> Saturation/1, Switch/3, Switch/2
  Simulation 3D Joystick/2 -> Rate Transition/1
  Saturation/1 -> PointToGo/2(In1)  "UserChoice"
  Demux1/1 -> Bus Creator/1  "u_x_raw"
  Demux1/3 -> Bus Creator/3  "u_r_raw"
  Simulation 3D Joystick/1 -> Rate Transition1/1
  Rate Transition/1 -> Selector2/1, Selector/1
  Rate Transition1/1 -> Selector1/1
  Rate Transition2/1 -> Display2/1
  Selector/1 -> Demux/1
  Demux/5 -> Hold/1(In1)
  Selector1/1 -> Demux1/1
  Selector2/1 -> Hold1/1(In1)  "AutoON"
  Hold1/1(Out1) -> Out1/1
  PointToGo/1(Out1) -> Out2/1
  Y_IN/1 -> PointToGo/1(Y_IN)
  Constant/1 -> Switch/1
  Switch/1 -> Out5/1  "ManualON"
  Demux/1 -> MissionNum/1(In1)  "One"
  Demux/2 -> MissionNum/2(In2)  "Two"
  Demux/3 -> MissionNum/3(In3)  "Three"
  Demux/4 -> MissionNum/4(In4)  "Four"
  Simulation 3D Joystick/3 -> Rate Transition2/1

== system Bossi_Emanuele_EE460S3D_R99/ControlLaw/Command/ManualMode ==
  ManualInput : Inport
  Trigger : Inport  Port=2
  CurrentPosition : Inport  Port=3
  CurrentVelocity : Inport  Port=4
  Action Port : ActionPort  ActionPortLabel=else
  Bus Creator : BusCreator  Inputs=9
  Bus Creator1 : BusCreator  Inputs=9
  Bus Creator2 : BusCreator  Inputs=6
  Bus Selector : BusSelector  OutputSignals=u_x_raw,u_y_raw,u_r_raw
  Bus Selector1 : BusSelector  OutputSignals=x_cmd,y_cmd,theta_cmd,xdot_cmd,ydot_cmd,theta_dot_cmd,xddot_cmd,yddot_cmd,theta_ddot_cmd
  Bus Selector2 : BusSelector  OutputSignals=u_x_raw,TriggeredPosition,TriggeredVelocity,Trigger,u_y_raw,TriggeredPosition,TriggeredVelocity,Trigger,u_r_raw,TriggeredPosition,TriggeredVelocity,Trigger
  Gain{,1..8} (9 alike) : Gain
  Selector : Selector  InputPortWidth=3  IndexOptions=Index vector (dialog)  Indices=[1]  OutputSizes=1
  Selector1 : Selector  InputPortWidth=3  IndexOptions=Index vector (dialog)  Indices=[3]  OutputSizes=1
  Selector2 : Selector  InputPortWidth=3  IndexOptions=Index vector (dialog)  Indices=[3]  OutputSizes=1
  Selector3 : Selector  InputPortWidth=3  IndexOptions=Index vector (dialog)  Indices=[2]  OutputSizes=1
  Selector4 : Selector  InputPortWidth=3  IndexOptions=Index vector (dialog)  Indices=[2]  OutputSizes=1
  Selector5 : Selector  InputPortWidth=3  IndexOptions=Index vector (dialog)  Indices=[1]  OutputSizes=1
  Theta_cmd : Subsystem
  X_cmd : Subsystem
  Y_cmd : Subsystem
  Out1 : Outport
  wires:
  Bus Creator1/1 -> Out1/1  "CMD"
  ManualInput/1 -> Bus Selector/1  "ManualInput"
  X_cmd/1(Out1) -> Bus Creator/1
  X_cmd/2(Out2) -> Bus Creator/2
  X_cmd/3(Out3) -> Bus Creator/3
  Y_cmd/1(Out1) -> Bus Creator/4
  Y_cmd/2(Out2) -> Bus Creator/5
  Y_cmd/3(Out3) -> Bus Creator/6
  Theta_cmd/1(Out1) -> Bus Creator/7
  Theta_cmd/2(Out2) -> Bus Creator/8
  Theta_cmd/3(Out3) -> Bus Creator/9
  Bus Creator/1 -> Bus Selector1/1  "CMD"
  Bus Selector1/1 -> Gain/1  "<x_cmd>"
  Bus Selector1/2 -> Gain1/1  "<y_cmd>"
  Bus Selector1/3 -> Gain2/1  "<theta_cmd>"
  Bus Selector1/4 -> Gain3/1  "<xdot_cmd>"
  Bus Selector1/5 -> Gain4/1  "<ydot_cmd>"
  Bus Selector1/6 -> Gain5/1  "<theta_dot_cmd>"
  Bus Selector1/7 -> Gain6/1  "<xddot_cmd>"
  Bus Selector1/8 -> Gain7/1  "<yddot_cmd>"
  Bus Selector1/9 -> Gain8/1  "<theta_ddot_cmd>"
  Gain/1 -> Bus Creator1/1
  Gain1/1 -> Bus Creator1/2
  Gain2/1 -> Bus Creator1/3
  Gain3/1 -> Bus Creator1/4
  Gain4/1 -> Bus Creator1/5
  Gain5/1 -> Bus Creator1/6
  Gain6/1 -> Bus Creator1/7
  Gain7/1 -> Bus Creator1/8
  Gain8/1 -> Bus Creator1/9
  Bus Selector/1 -> Bus Creator2/1  "<u_x_raw>"
  Bus Selector/2 -> Bus Creator2/2  "<u_y_raw>"
  Bus Selector/3 -> Bus Creator2/3  "<u_r_raw>"
  Bus Creator2/1 -> Bus Selector2/1
  CurrentPosition/1 -> Bus Creator2/4
  CurrentVelocity/1 -> Bus Creator2/5
  Trigger/1 -> Bus Creator2/6
  Bus Selector2/1 -> X_cmd/1(In1)  "<u_x_raw>"
  Bus Selector2/2 -> Selector/1  "<TriggeredPosition>"
  Bus Selector2/3 -> Selector5/1  "<TriggeredVelocity>"
  Bus Selector2/4 -> X_cmd/4(In2), X_cmd/5(In4)  "<Trigger>"
  Bus Selector2/5 -> Y_cmd/1(In1)  "<u_y_raw>"
  Bus Selector2/6 -> Selector3/1  "<TriggeredPosition>"
  Bus Selector2/7 -> Selector4/1  "<TriggeredVelocity>"
  Bus Selector2/8 -> Y_cmd/5(In5), Y_cmd/4(In2)  "<Trigger>"
  Bus Selector2/9 -> Theta_cmd/1(In1)  "<u_r_raw>"
  Bus Selector2/10 -> Selector1/1  "<TriggeredPosition>"
  Bus Selector2/11 -> Selector2/1  "<TriggeredVelocity>"
  Bus Selector2/12 -> Theta_cmd/5(In5), Theta_cmd/4(In2)  "<Trigger>"
  Selector/1 -> X_cmd/2(In5)  "Xpos"
  Selector5/1 -> X_cmd/3(In3)  "Xvel"
  Selector3/1 -> Y_cmd/2(In4)  "Yposl"
  Selector4/1 -> Y_cmd/3(In3)  "Yvel"
  Selector1/1 -> Theta_cmd/2(In4)  "Rpos"
  Selector2/1 -> Theta_cmd/3(In3)  "Rvel"

== system Bossi_Emanuele_EE460S3D_R99/ControlLaw/Command/Trigger1 ==
  In2 : Inport
  In1 : Inport  Port=2
  Bus Creator1 : BusCreator  Inputs=3
  Bus Creator2 : BusCreator  Inputs=3
  Bus Selector4 : BusSelector  OutputSignals=Xpos_m,Ypos_m,theta_pos_deg
  Bus Selector5 : BusSelector  OutputSignals=AutoON,positions
  Constant : Constant  Value=Pdata  SampleTime=dt
  PositionTrigger : Subsystem  TreatAsAtomicUnit=on
  TriggerCondition : Subsystem
  Trigger : Outport
  Out1 : Outport  Port=2
  wires:
  Bus Selector4/3 -> Bus Creator2/3  "<theta_pos_deg>"
  Bus Selector5/1 -> TriggerCondition/1(In2)  "<AutoON>"
  TriggerCondition/1(Trigger) -> Trigger/1, PositionTrigger/Trigger
  Constant/1 -> Bus Creator1/2  "Pdata"
  Bus Creator1/1 -> Bus Selector5/1
  Bus Selector4/1 -> Bus Creator2/1  "<Xpos_m>"
  Bus Selector4/2 -> Bus Creator2/2  "<Ypos_m>"
  Bus Selector5/2 -> PositionTrigger/1(In1)  "<positions>"
  In2/1 -> Bus Creator1/1
  In1/1 -> Bus Selector4/1
  Bus Creator2/1 -> Bus Creator1/3  "positions"
  PositionTrigger/1(CurrentPosition1) -> Out1/1  "TriggeredPosition"

== system Bossi_Emanuele_EE460S3D_R99/ControlLaw/Command/Trigger2 ==
  In2 : Inport
  In1 : Inport  Port=2
  Bus Creator : BusCreator  Inputs=2
  Bus Creator1 : BusCreator  Inputs=4
  Bus Creator2 : BusCreator  Inputs=3
  Bus Creator3 : BusCreator  Inputs=3
  Bus Selector : BusSelector  OutputSignals=Trigger,velocities
  Bus Selector1 : BusSelector  OutputSignals=Xvel_mps,Yvel_mps,theta_vel_degps
  Bus Selector4 : BusSelector  OutputSignals=Xpos_m,Ypos_m,theta_pos_deg
  Bus Selector5 : BusSelector  OutputSignals=velocities,ManualMode,positions
  Constant : Constant  Value=Pdata  SampleTime=dt
  PositionTrigger : Subsystem  TreatAsAtomicUnit=on
  TriggerCondition : Subsystem
  VelocityTrigger : Subsystem  TreatAsAtomicUnit=on
  Trigger : Outport
  TriggeredPosition : Outport  Port=2
  TriggeredVelocity : Outport  Port=3
  wires:
  Bus Selector4/3 -> Bus Creator2/3  "<theta_pos_deg>"
  Bus Selector5/2 -> TriggerCondition/1(In2)  "<ManualMode>"
  TriggerCondition/1(Trigger) -> Bus Creator/2, PositionTrigger/Trigger, Trigger/1
  Constant/1 -> Bus Creator1/2  "Pdata"
  Bus Creator1/1 -> Bus Selector5/1
  Bus Selector4/1 -> Bus Creator2/1  "<Xpos_m>"
  Bus Selector4/2 -> Bus Creator2/2  "<Ypos_m>"
  Bus Selector5/3 -> PositionTrigger/1(In1)  "<positions>"
  In2/1 -> Bus Creator1/1
  In1/1 -> Bus Selector1/1, Bus Selector4/1
  Bus Creator2/1 -> Bus Creator1/3  "positions"
  PositionTrigger/1(CurrentPosition1) -> TriggeredPosition/1  "TriggeredPosition"
  Bus Selector1/3 -> Bus Creator3/3  "<theta_vel_degps>"
  Bus Selector1/1 -> Bus Creator3/1  "<Xvel_mps>"
  Bus Selector1/2 -> Bus Creator3/2  "<Yvel_mps>"
  Bus Creator3/1 -> Bus Creator1/4  "velocities"
  Bus Selector5/1 -> Bus Creator/1  "<velocities>"
  Bus Creator/1 -> Bus Selector/1
  Bus Selector/2 -> VelocityTrigger/1(In1)  "<velocities>"
  Bus Selector/1 -> VelocityTrigger/Trigger  "<Trigger>"
  VelocityTrigger/1(CurrentVelocity) -> TriggeredVelocity/1  "TriggeredVelocity"
